simulink model "NonIsolatedDCDCTestHarnessPlant"  (R2026a)
settings: Solver=ode23t  StopTime=0.02  MaxStep=1e-5  AbsTol=1e-3
PreLoadFcn:
  | NonIsolatedDCDCDefaultInputParameters;
model workspace (MAT data in the model file):
  ConverterKey = "NonIsolatedDCDC"
undefined symbols (not defined in the file or in its folder): DiscIntNeverNeededParam, nonIsolatedDCDCController
libraries: nesl_utility x47, ee_lib x43, fl_lib x42
(part 1 of 5)
settings Model: Creator=vsolaise  LastModifiedBy=vsolaise
settings SimscapeCC: SimscapeNominalValues="[{\"value\":\"1\",\"unit\":\"A\"},{\"value\":\"1\",\"unit\":\"bar\"},{\"value\":\"1\",\"unit\":\"cm^2\"},{\"value\":\"1\",\"unit\":\"cm^3/s\"},{\"value\":\"1\",\"unit\":\"kJ/kg\"},{\"value\":\"1\",\"unit\":\"kW\"},{\"value\":\"1\",\"unit\":\"l\"},{\"value\":\"1\",\"unit\":\"N\"},{\"value\":\"1\",\"unit\":\"N*m\"},{\"value\":\"1\",\"unit\":\"V\"}]"  SimscapeLogDataHistory=5000.0

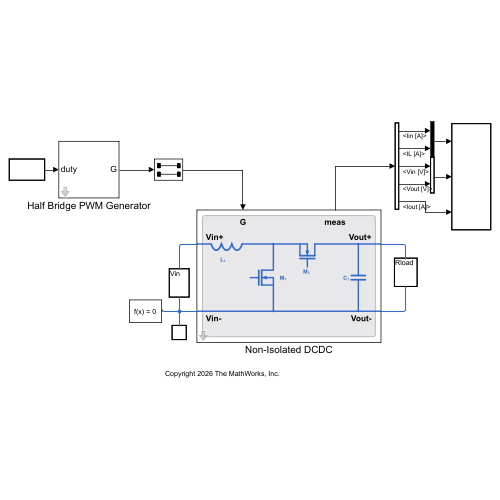
[thumbnail: Simulink's stored preview of the top-level diagram]
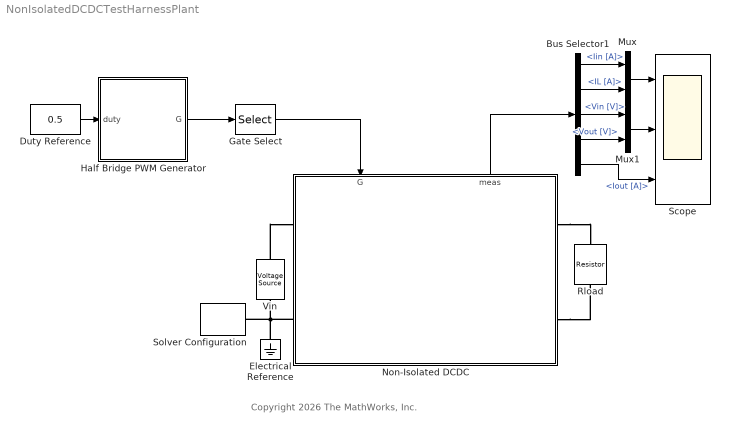
== system NonIsolatedDCDCTestHarnessPlant ==
  note: Copyright 2026 The MathWorks, Inc.
  Bus Selector1 : BusSelector  OutputSignals=Iin [A],IL [A],Vin [V],Vout [V],Iout [A]
  Duty Reference : Constant  Value=0.5
  Electrical Reference : fl_lib/Electrical/Electrical Elements/Electrical Reference
  Gate Select : Selector  InputPortWidth=2  IndexOptions=Index vector (dialog)  Indices=[1 2]  OutputSizes=1
  Half Bridge PWM Generator : Subsystem  mask(Half Bridge PWM Generator){solverMode=Variable-step (continuous), Ts=1e-8, Fsw=nonIsolatedDCDCController.Fsw.value, Tdead=nonIsolatedDCDCController.Tdead.value, gateVoltageOn=nonIsolatedDCDCController.gateVoltageOn.value, gateVoltageOff=nonIsolatedDCDCController.gateVoltageOff.value}
      mask prompts: solverMode "Solver mode"; Ts "Sample time (s)"; Fsw "Switching frequency (Hz)"; Tdead "Dead time (s)"; gateVoltageOn "Gate ON voltage (V)"; gateVoltageOff "Gate OFF voltage (V)"
      mask help:
      | This block generates half-bridge PWM gate signals with a dead time from a commanded duty cycle.
      |
      | For a variable-step solver, set Solver mode to Variable-step (continuous). For a fixed-step solver, set Solver mode to Fixed-step (discrete) and set Sample time to a positive value.
      mask init:
      | % Solver mode. Switch every sawtooth ramp in this block between its continuous
      | % and its discrete implementation, and show the sample time only when it is used.
      | pwmGeneratorBlock = gcb;
      | if strcmp(get_param(pwmGeneratorBlock, 'solverMode'), 'Fixed-step (discrete)')
      |     pwmGeneratorRampChoice = 'FixedStep';
      |     pwmGeneratorSampleTimeVisibility = 'on';
      | else
      |     pwmGeneratorRampChoice = 'VariableStep';
      |     pwmGeneratorSampleTimeVisibility = 'off';
      | end
      | 
      | % A block may hold more than one ramp, at any depth, so the ramps are found by the
      | % "Ramp Mode" suffix on their names rather than by one fixed path. The match filter
      | % keeps every variant choice in the search, which is also what silences the
      | % find_system default-variants warning.
      | pwmGeneratorRamps = find_system(pwmGeneratorBlock, ...
      |     'MatchFilter', @Simulink.match.allVariants, 'LookUnderMasks', 'all', ...
      |     'FollowLinks', 'on', 'Regexp', 'on', 'BlockType', 'SubSystem', ...
      |     'Name', 'Ramp Mode$');
      | for pwmGeneratorRampIndex = 1:numel(pwmGeneratorRamps)
      |     set_param(pwmGeneratorRamps{pwmGeneratorRampIndex}, ...
      |         'LabelModeActiveChoice', pwmGeneratorRampChoice);
      | end
      | 
      | % Only the discrete ramp declares a rate, so the sample time is hidden in the
      | % continuous mode. The guard keeps the code silent on a mask still being built.
      | pwmGeneratorMask = Simulink.Mask.get(pwmGeneratorBlock);
      | pwmGeneratorSampleTime = pwmGeneratorMask.getParameter('Ts');
      | if ~isempty(pwmGeneratorSampleTime)
      |     pwmGeneratorSampleTime.Visible = pwmGeneratorSampleTimeVisibility;
      | end
      mask Help: web('HalfBridgePWMGenerator.html')
      mask TypeOptions solverMode: Variable-step (continuous) | Fixed-step (discrete)
      mask Callback solverMode:
      | % Solver mode. Switch every sawtooth ramp in this block between its continuous
      | % and its discrete implementation, and show the sample time only when it is used.
      | pwmGeneratorBlock = gcb;
      | if strcmp(get_param(pwmGeneratorBlock, 'solverMode'), 'Fixed-step (discrete)')
      |     pwmGeneratorRampChoice = 'FixedStep';
      |     pwmGeneratorSampleTimeVisibility = 'on';
      | else
      |     pwmGeneratorRampChoice = 'VariableStep';
      |     pwmGeneratorSampleTimeVisibility = 'off';
      | end
      | 
      | % A block may hold more than one ramp, at any depth, so the ramps are found by the
      | % "Ramp Mode" suffix on their names rather than by one fixed path. The match filter
      | % keeps every variant choice in the search, which is also what silences the
      | % find_system default-variants warning.
      | pwmGeneratorRamps = find_system(pwmGeneratorBlock, ...
      |     'MatchFilter', @Simulink.match.allVariants, 'LookUnderMasks', 'all', ...
      |     'FollowLinks', 'on', 'Regexp', 'on', 'BlockType', 'SubSystem', ...
      |     'Name', 'Ramp Mode$');
      | for pwmGeneratorRampIndex = 1:numel(pwmGeneratorRamps)
      |     set_param(pwmGeneratorRamps{pwmGeneratorRampIndex}, ...
      |         'LabelModeActiveChoice', pwmGeneratorRampChoice);
      | end
      | 
      | % Only the discrete ramp declares a rate, so the sample time is hidden in the
      | % continuous mode. The guard keeps the code silent on a mask still being built.
      | pwmGeneratorMask = Simulink.Mask.get(pwmGeneratorBlock);
      | pwmGeneratorSampleTime = pwmGeneratorMask.getParameter('Ts');
      | if ~isempty(pwmGeneratorSampleTime)
      |     pwmGeneratorSampleTime.Visible = pwmGeneratorSampleTimeVisibility;
      | end
      mask DialogControl DescTextVar Prompt:
      | This block generates half-bridge PWM gate signals with a dead time from a commanded duty cycle.
      | 
      | For a variable-step solver, set Solver mode to Variable-step (continuous). For a fixed-step solver, set Solver mode to Fixed-step (discrete) and set Sample time to a positive value.
      mask DialogControl SolverPanel Prompt: Solver Settings
      mask DialogControl SwitchingPanel Prompt: Switching Parameters
      mask DialogControl GateDrivePanel Prompt: Gate Drive
  Mux : Mux  Inputs=2
  Mux1 : Mux  Inputs=2
  Non-Isolated DCDC : Subsystem  mask(Non-Isolated DC-DC Converter){modelOption=Synchronous Boost, ratedPower=1500, ratedPower_unit=W, Vin=200, Vin_unit=V, Vout=400, Vout_unit=V, Fsw=100000, Fsw_unit=Hz, L=4.356e-4, L_unit=H, RL=0.05, RL_unit=Ohm, C=1.8651e-4, C_unit=F, Rco=0.02, Rco_unit=Ohm, Vco=320, Vco_unit=V, switchDeviceOption=MOSFET (Ideal, Switching) with Thermal, RdsOn=0.02, RdsOn_unit=Ohm, GdsOff=1e-8, GdsOff_unit=1/Ohm, Vth=0.5, Vth_unit=V, VfBody=2.04, VfBody_unit=V, RdBody=0.004, RdBody_unit=Ohm, GdBody=1e-6, GdBody_unit=1/Ohm, diodeDeviceOption=Ideal Diode, Vf=0.5, Vf_unit=V, Rd=0.01, Rd_unit=Ohm, Gd=1e-8, Gd_unit=1/Ohm, simTemp=25, simTemp_unit=degC}
      mask prompts: modelOption "Topology"; ratedPower "Rated power"; Vin "Input voltage"; Vout "Output voltage"; Fsw "Switching frequency"; L "Inductance"; RL "Inductor resistance"; C "Output capacitance"; Rco "Capacitor ESR"; Vco "Initial output capacitor voltage"; switchDeviceOption "Main switch device"; RdsOn "On-state resistance"; GdsOff "Off-state conductance"; Vth "Threshold voltage"; VfBody "Body diode forward voltage"; RdBody "Body diode on resistance"; GdBody "Body diode off conductance"; diodeDeviceOption "Diode device"; Vf "Diode forward voltage"; Rd "Diode on resistance"; Gd "Diode off conductance"; simTemp "Simulation temperature"
      mask help: Buck, Boost, or Buck-Boost DC-DC converter with optional synchronous rectification
      mask init:
      | %% Unit conversion: convert displayed values to base SI units
      | convMap = containers.Map( ...
      |     {'W','kW','MW','V','kV','mV','F','mF','uF','nF','pF', ...
      |      'H','mH','uH','nH','Ohm','kOhm','mOhm','S','mS','1/Ohm', ...
      |      'Hz','kHz','MHz'}, ...
      |     {1, 1e3, 1e6, 1, 1e3, 1e-3, 1, 1e-3, 1e-6, 1e-9, 1e-12, ...
      |      1, 1e-3, 1e-6, 1e-9, 1, 1e3, 1e-3, 1, 1e-3, 1, ...
      |      1, 1e3, 1e6});
      | 
      | ratedPower_SI = ratedPower * convMap(ratedPower_unit);
      | Vin_SI = Vin * convMap(Vin_unit);
      | Vout_SI = Vout * convMap(Vout_unit);
      | Fsw_SI = Fsw * convMap(Fsw_unit);
      | L_SI = L * convMap(L_unit);
      | RL_SI = RL * convMap(RL_unit);
      | C_SI = C * convMap(C_unit);
      | Rco_SI = Rco * convMap(Rco_unit);
      | Vco_SI = Vco * convMap(Vco_unit);
      | RdsOn_SI = RdsOn * convMap(RdsOn_unit);
      | GdsOff_SI = GdsOff * convMap(GdsOff_unit);
      | Vth_SI = Vth * convMap(Vth_unit);
      | Vf_SI = Vf * convMap(Vf_unit);
      | Rd_SI = Rd * convMap(Rd_unit);
      | Gd_SI = Gd * convMap(Gd_unit);
      | VfBody_SI = VfBody * convMap(VfBody_unit);
      | RdBody_SI = RdBody * convMap(RdBody_unit);
      | GdBody_SI = GdBody * convMap(GdBody_unit);
      | 
      | %% Simulation temperature
      | % Temperature is an offset unit (K = degC + 273.15), so it cannot use convMap.
      | % simTemp_K is read by the thermal MOSFET junction target and Temperature Source,
      | % and by the tabulated diode device temperature.
      | if strcmp(simTemp_unit, 'degC')
      |     simTemp_K = simTemp + 273.15;
      | else
      |     simTemp_K = simTemp;
      | end
      | 
      | %% Apply variant selection
      | selectDCDCModelOption(gcb);
      settings: CopyFcn="set_param(gcbh,\"LinkStatus\",\"none\");"  PortSchema="{\"entries\":[{\"content\":{\"sides\":[{\"content\":{\"connectorIds\":[\"LConn1\",\"LConn2\"]},\"type\":\"ConnectorPlacement.EquallySpacedRectSide\",\"uuid\":\"902a8dfc-7104-4c05-856d-94df839e3447\"},{\"content\":{\"connectorIds\":[\"RConn1\",\"RConn2\"],\"side\":\"RIGHT\"},\"type\":\"ConnectorPlacement.EquallySpacedRectSide\",\"uuid\":\"60097652-723c-4c8b-adb2-e2e896cce9b8\"},{\"content\":{\"connectorIds\":[\"In1\",\"Out1\"],\"side\":\"TOP\"},\"type\":\"ConnectorPlacement.EquallySpacedRectSide\",\"uuid\":\"37713e19-e822-434b-b66d-56986e674464\"}]},\"type\":\"ConnectorPlacement.EquallySpacedConnector\",\"uuid\":\"e0b4e08f-2e15-4704-9b91-0fcfb097a2d4\"}],\"packageUris\":[\"http://schema.mathworks.com/mf0/Connector/R2020b\"],\"version\":\"1.0\"}"
      mask Help: web('NonIsolatedDCDC.html')
      mask TypeOptions modelOption: Buck | Synchronous Buck | Boost | Synchronous Boost | Buck-Boost | Synchronous Buck-Boost
      mask Callback modelOption: selectDCDCModelOption(gcb);
      mask TypeOptions ratedPower_unit: W | kW | MW
      mask TypeOptions Vin_unit: V | mV | kV
      mask TypeOptions Vout_unit: V | mV | kV
      mask TypeOptions Fsw_unit: Hz | kHz | MHz
      mask TypeOptions L_unit: H | mH | uH | nH
      mask TypeOptions RL_unit: Ohm | mOhm
      mask TypeOptions C_unit: F | mF | uF | nF | pF
      mask TypeOptions Rco_unit: Ohm | mOhm
      mask TypeOptions Vco_unit: V | kV | mV
      mask TypeOptions switchDeviceOption: Ideal Switch | MOSFET (Ideal, Switching) with Thermal
      mask Callback switchDeviceOption: selectDCDCMainSwitch(gcb);
      mask TypeOptions RdsOn_unit: Ohm | mOhm
      mask TypeOptions GdsOff_unit: 1/Ohm | S
      mask TypeOptions Vth_unit: V | mV
      mask TypeOptions VfBody_unit: V | mV
      mask TypeOptions RdBody_unit: Ohm | mOhm
      mask TypeOptions GdBody_unit: 1/Ohm | S
      mask TypeOptions diodeDeviceOption: Ideal Diode | Tabulated Diode
      mask Callback diodeDeviceOption: selectDCDCDiodeDevice(gcb);
      mask TypeOptions Vf_unit: V | mV
      mask TypeOptions Rd_unit: Ohm | mOhm
      mask TypeOptions Gd_unit: 1/Ohm | S
      mask TypeOptions simTemp_unit: degC | K
      mask DialogControl DC_DCConverterParameters Prompt: DC-DC Converter Parameters
      mask DialogControl SwitchDevice Prompt: Switch Device
      mask DialogControl openMOSFETMask Prompt: Open MOSFET block mask
      mask DialogControl openMOSFETMask Callback: openDCDCMOSFETMask(gcb);
      mask DialogControl DiodeDevice Prompt: Diode Device
      mask DialogControl openDiodeMask Prompt: Open Diode block mask
      mask DialogControl openDiodeMask Callback: openDCDCDiodeMask(gcb);
      mask DialogControl ExportPanel Prompt: Export to Unmasked Subsystem
      mask DialogControl ExportInfo Prompt: To customize the converter, export it as an unmasked subsystem with the active variant flattened - a standalone, fully-editable circuit plus a parameter file. Requires the "Variant Manager for Simulink" add-on.
      mask DialogControl exportToModel Prompt: Export
      mask DialogControl exportToModel Callback: exportConverterModelFromMask(gcb);
      mask Display:
      | topology = get_param(gcb, 'modelOption');
      | if strcmp(topology, 'Buck')
      |     image('BuckDiodeIcon.svg');
      | elseif strcmp(topology, 'Synchronous Buck')
      |     image('BuckSyncMOSIcon.svg');
      | elseif strcmp(topology, 'Boost')
      |     image('BoostDiodeIcon.svg');
      | elseif strcmp(topology, 'Synchronous Boost')
      |     image('BoostSyncMOSIcon.svg');
      | elseif strcmp(topology, 'Buck-Boost')
      |     image('BuckBoostDiodeIcon.svg');
      | else
      |     image('BuckBoostSyncMOSIcon.svg');
      | end
  Rload : fl_lib/Electrical/Electrical Elements/Resistor  R=106.667 Ohm  i_specify=off  i_priority=None  i=0 A  i_nominal_specify=off  i_nominal_value=1  i_nominal_unit=A  v_specify=off  v_priority=None  v=0 V  v_nominal_specify=off  v_nominal_value=1  v_nominal_unit=V
  Scope : Scope  NumInputPorts=3
      settings: ActiveDisplayString=3  Title=Output Current (A)  ActiveDisplayYMinimum=2.82510959569979  ActiveDisplayYMaximum=4.5280130894318766
  Solver Configuration : nesl_utility/Solver Configuration  PhysicalDomain=network_engine_domain  SubClassName=solver  LeftPortType=input  RightPortType=generic  Tones=[]  Harmonics=[]  SimulateNoise=off  Profile=off  UseLocalSampling=off  EnableSwitchedLinearOptims=on  FrequencyDomain=off  UseCCode=off  RelTol=0.001  AbsTol=0.001  MinStep=1e-09  ToWorkspace=off  RevertToSquareIcSolve=off  NumHomotopyIterations=100  PhasorMode=off  PhasorModeNumHarmonics=1  ConsistencySolver=NEWTON_XTOL_AFTER_FTOL  CanonicalOrdering=UNORDERED  OptimizeIntermediates=UNOPTIMIZED  IndexReductionMethod=DerivativeReplacement  DoDC=off  ResidualTolerance=1e-09  ConsistencyTolSource=GLOBAL  ConsistencyAbsTol=0.001  ConsistencyRelTol=0.001  ConsistencyTolFactor=0.001  UseLocalSolver=on  LocalSolverChoice=NE_BACKWARD_EULER_ADVANCER  ResolveIndetEquations=on  FunctionEvalNumThread=1  LocalSolverSampleTime=2e-7  DoFixedCost=on  MaxNonlinIter=3  MaxModeIter=2  ComputeImpulses=off  ImpulseIterations=2  LinearAlgebra=auto  LinearAlgebraNumThread=0  EquationFormulation=NE_TIME_EF  DelaysMemoryBudget=1024  AutomaticFiltering=on  FilteringTimeConstant=0.001  PartitionStorageMethod=AS_NEEDED  PartitionMemoryBudget=1024  PartitionMethod=ROBUST  MultibodyUseLocalSolver=off  MultibodyLocalSolverChoice=ODE1  MultibodyLocalSolverSampleTime=0.001
  Vin : ee_lib/Sources/Voltage Source  dc_voltage=200 V  ac_voltage=0 V  ac_shift=0 rad  ac_frequency=60 Hz  noise_mode=ee.enum.sources.noise.Disabled  PSD=0 V^2/Hz  sample_time=1e-3 s  repeatability=ee.enum.sources.repeatability.NotRepeatable  user_seed=0  auto_seed=4267928862  i_specify=off  i_priority=None  i=0 A  i_nominal_specify=off  i_nominal_value=1  i_nominal_unit=A  v_specify=off  v_priority=None  v=0 V  v_nominal_specify=off  v_nominal_value=1  v_nominal_unit=V
  wires:
  Non-Isolated DCDC/1(meas) -> Bus Selector1/1
  Bus Selector1/2 -> Mux/2  "<IL [A]>"
  Bus Selector1/1 -> Mux/1  "<Iin [A]>"
  Bus Selector1/3 -> Mux1/1  "<Vin [V]>"
  Bus Selector1/4 -> Mux1/2  "<Vout [V]>"
  Mux1/1 -> Scope/2
  Mux/1 -> Scope/1
  Bus Selector1/5 -> Scope/3  "<Iout [A]>"
  Duty Reference/1 -> Half Bridge PWM Generator/1(duty)
  Half Bridge PWM Generator/1(G) -> Gate Select/1
  Gate Select/1 -> Non-Isolated DCDC/1(G)
  connections:
  Vin/LConn1 -- Non-Isolated DCDC/LConn1
  Non-Isolated DCDC/RConn1 -- Rload/LConn1
  Non-Isolated DCDC/RConn2 -- Rload/RConn1
  Electrical Reference/LConn1 -- Solver Configuration/RConn1 -- Non-Isolated DCDC/LConn2 -- Vin/RConn1

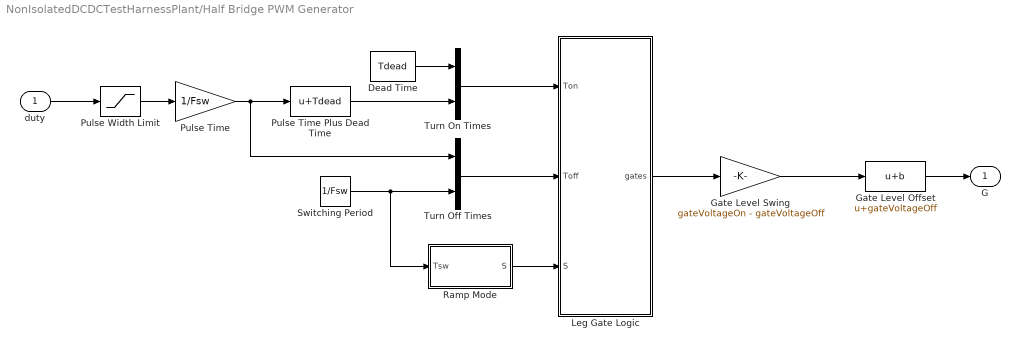
== system NonIsolatedDCDCTestHarnessPlant/Half Bridge PWM Generator ==
  duty : Inport
  Dead Time : Constant  Value=Tdead
  Gate Level Offset : Bias  Bias=gateVoltageOff
  Gate Level Swing : Gain  Gain=gateVoltageOn - gateVoltageOff
  Leg Gate Logic : Subsystem
  Pulse Time : Gain  Gain=1/Fsw
  Pulse Time Plus Dead Time : Bias  Bias=Tdead
  Pulse Width Limit : Saturate  UpperLimit=1 - Tdead*Fsw  LowerLimit=Tdead*Fsw
  Ramp Mode : Subsystem  Variant=on  VariantControlMode=label  LabelModeActiveChoice=VariableStep
  Switching Period : Constant  Value=1/Fsw
  Turn Off Times : Mux  Inputs=2
  Turn On Times : Mux  Inputs=2
  G : Outport
  wires:
  Gate Level Offset/1 -> G/1
  Leg Gate Logic/1(gates) -> Gate Level Swing/1
  Ramp Mode/1(S) -> Leg Gate Logic/3(S)
  Turn Off Times/1 -> Leg Gate Logic/2(Toff)
  Turn On Times/1 -> Leg Gate Logic/1(Ton)
  Gate Level Swing/1 -> Gate Level Offset/1
  Switching Period/1 -> Ramp Mode/1(Tsw), Turn Off Times/2
  Pulse Time Plus Dead Time/1 -> Turn On Times/2
  Dead Time/1 -> Turn On Times/1
  Pulse Time/1 -> Turn Off Times/1, Pulse Time Plus Dead Time/1
  Pulse Width Limit/1 -> Pulse Time/1
  duty/1 -> Pulse Width Limit/1

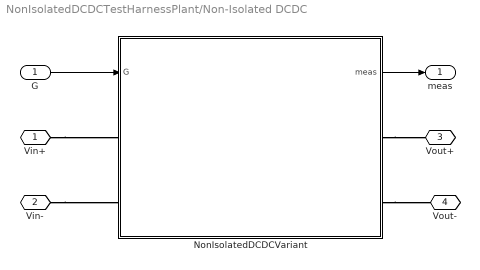
== system NonIsolatedDCDCTestHarnessPlant/Non-Isolated DCDC ==
  G : Inport
  NonIsolatedDCDCVariant : Subsystem  Variant=on  VariantControlMode=label  LabelModeActiveChoice=SynchronousBoost
  Vin+ : PMIOPort  Side=Left
  Vin- : PMIOPort  Port=2  Side=Left
  Vout+ : PMIOPort  Port=3  Side=Right
  Vout- : PMIOPort  Port=4  Side=Right
  meas : Outport
  wires:
  NonIsolatedDCDCVariant/1(meas) -> meas/1
  G/1 -> NonIsolatedDCDCVariant/1(G)
  connections:
  NonIsolatedDCDCVariant/RConn2 -- Vout-/RConn1
  NonIsolatedDCDCVariant/RConn1 -- Vout+/RConn1
  Vin-/RConn1 -- NonIsolatedDCDCVariant/LConn2
  Vin+/RConn1 -- NonIsolatedDCDCVariant/LConn1

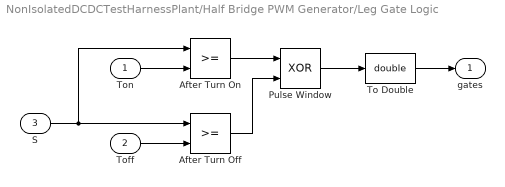
== system NonIsolatedDCDCTestHarnessPlant/Half Bridge PWM Generator/Leg Gate Logic ==
  Ton : Inport
  Toff : Inport  Port=2
  S : Inport  Port=3
  After Turn Off : RelationalOperator
  After Turn On : RelationalOperator
  Pulse Window : Logic  Operator=XOR
  To Double : DataTypeConversion  OutDataTypeStr=double
  gates : Outport
  wires:
  To Double/1 -> gates/1
  Pulse Window/1 -> To Double/1
  After Turn Off/1 -> Pulse Window/2
  After Turn On/1 -> Pulse Window/1
  S/1 -> After Turn On/1, After Turn Off/1
  Toff/1 -> After Turn Off/2
  Ton/1 -> After Turn On/2

== system NonIsolatedDCDCTestHarnessPlant/Half Bridge PWM Generator/Ramp Mode ==
  Tsw : Inport
  FixedStep : Subsystem  VariantControl=FixedStep
  VariableStep : Subsystem  VariantControl=VariableStep
  S : Outport

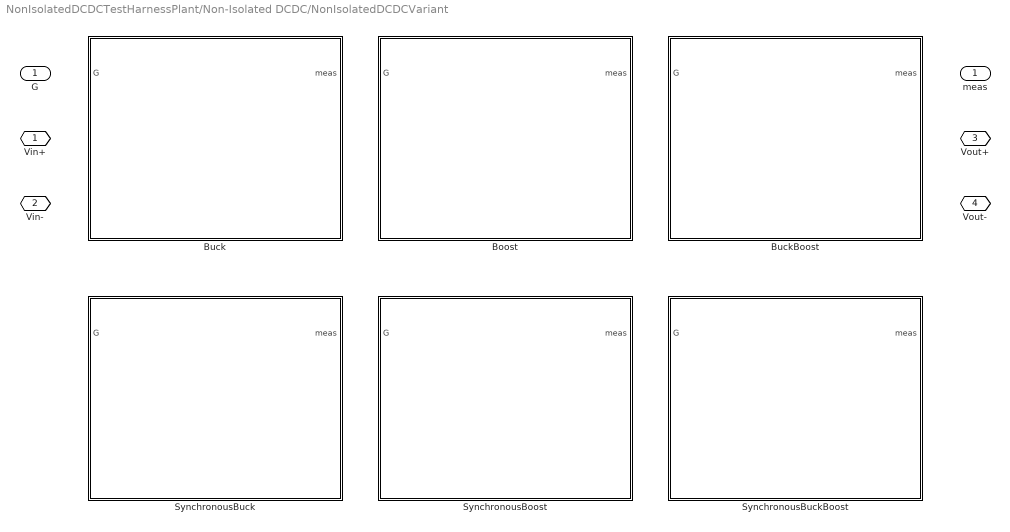
== system NonIsolatedDCDCTestHarnessPlant/Non-Isolated DCDC/NonIsolatedDCDCVariant ==
  G : Inport
  Boost : Subsystem  VariantControl=Boost
  Buck : Subsystem  VariantControl=Buck
  BuckBoost : Subsystem  VariantControl=BuckBoost
  SynchronousBoost : Subsystem  VariantControl=SynchronousBoost
  SynchronousBuck : Subsystem  VariantControl=SynchronousBuck
  SynchronousBuckBoost : Subsystem  VariantControl=SynchronousBuckBoost
  Vin+ : PMIOPort  Side=Left
  Vin- : PMIOPort  Port=2  Side=Left
  Vout+ : PMIOPort  Port=3  Side=Right
  Vout- : PMIOPort  Port=4  Side=Right
  meas : Outport

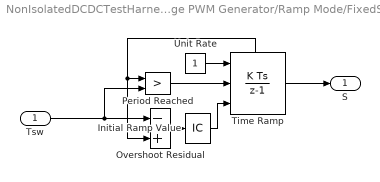
== system NonIsolatedDCDCTestHarnessPlant/Half Bridge PWM Generator/Ramp Mode/FixedStep ==
  Tsw : Inport
  Initial Ramp Value : InitialCondition  Value=0
  Overshoot Residual : Sum  Inputs=-+
  Period Reached : RelationalOperator  Operator=>  ZeroCross=off
  Time Ramp : DiscreteIntegrator  ExternalReset=rising  InitialConditionSource=external  SampleTime=Ts  ShowStatePort=on  ICPrevOutput=DiscIntNeverNeededParam  ICPrevScaledInput=DiscIntNeverNeededParam
  Unit Rate : Constant
  S : Outport
  wires:
  Initial Ramp Value/1 -> Time Ramp/3
  Overshoot Residual/1 -> Initial Ramp Value/1
  Time Ramp/State -> Overshoot Residual/2, Period Reached/1
  Tsw/1 -> Period Reached/2, Overshoot Residual/1
  Time Ramp/1 -> S/1
  Period Reached/1 -> Time Ramp/2
  Unit Rate/1 -> Time Ramp/1

== system NonIsolatedDCDCTestHarnessPlant/Half Bridge PWM Generator/Ramp Mode/VariableStep ==
  Tsw : Inport
  Initial Ramp Value : InitialCondition  Value=0
  Overshoot Residual : Sum  Inputs=-+
  Period Reached : RelationalOperator  Operator=>
  Time Ramp : Integrator  ExternalReset=rising  InitialConditionSource=external  ShowStatePort=on
  Unit Rate : Constant
  S : Outport
  wires:
  Initial Ramp Value/1 -> Time Ramp/3
  Overshoot Residual/1 -> Initial Ramp Value/1
  Time Ramp/State -> Overshoot Residual/2, Period Reached/1
  Tsw/1 -> Period Reached/2, Overshoot Residual/1
  Time Ramp/1 -> S/1
  Period Reached/1 -> Time Ramp/2
  Unit Rate/1 -> Time Ramp/1

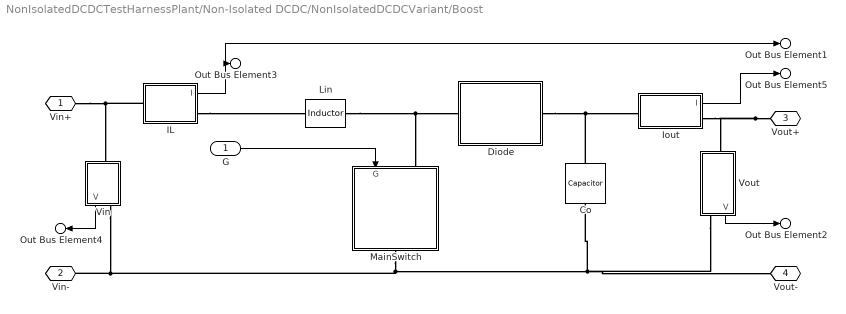
== system NonIsolatedDCDCTestHarnessPlant/Non-Isolated DCDC/NonIsolatedDCDCVariant/Boost ==
  G : Inport
  Co : ee_lib/Passive/Capacitor  cap_option=ee.enum.passive.capacitor.capOption.const  c=C_SI F  Cvec=[1e-05, 1e-06] F  Vvec=[0, 10] V  CV_table_symmetry=ee.enum.passive.capacitor.tableSymmetry.yes  f_vec=[1, 10] kHz  DFext_vec=[.8, 1.2]  enable_C_tol=ee.enum.toleranceApplication.none  averaging_period=0 s  C_tol=5  tol_distribution=ee.enum.toleranceDistribution.uniform  nSigma=4  r=Rco_SI Ohm  g=0 1/Ohm  enable_operating_limits=ee.enum.enable.no  operating_limit_action=ee.enum.passive.reportOpLim.warn  max_working_voltage_range=[-25, 25] V  power_rating=1 W  maxTemperature=85 degC  thermalEnable=false  thermalMass=1 J/K  i_specify=off  i_priority=None  i=0 A  i_nominal_specify=off  i_nominal_value=1  i_nominal_unit=A  v_specify=off  v_priority=None  v=0 V  v_nominal_specify=off  v_nominal_value=1  v_nominal_unit=V  vc_specify=on  vc_priority=High  vc=Vco_SI V  vc_nominal_specify=off  vc_nominal_value=1  vc_nominal_unit=V  T_specify=off  T_priority=None  T=298.15 K  T_nominal_specify=off  T_nominal_value=1  T_nominal_unit=K
  Diode : Subsystem  Variant=on  VariantControlMode=label  LabelModeActiveChoice=IdealDiode
  IL : Subsystem
      mask Display: disp('I')
  Iout : Subsystem
      mask Display: disp('I')
  Lin : ee_lib/Passive/Inductor  l=L_SI H  enable_L_tol=ee.enum.toleranceApplication.none  L_tol=20  tol_distribution=ee.enum.toleranceDistribution.uniform  nSigma=4  r=RL_SI Ohm  g=1e-9 1/Ohm  enable_operating_limits=ee.enum.enable.no  operating_limit_action=ee.enum.passive.reportOpLim.warn  max_working_current=1 A  power_rating=1 W  i_L_specify=off  i_L_priority=High  i_L=0 A  i_L_nominal_specify=off  i_L_nominal_value=1  i_L_nominal_unit=A
  MainSwitch : Subsystem  Variant=on  VariantControlMode=label  LabelModeActiveChoice=SwitchingMOSFETwithThermal
  Vin : Subsystem
      mask Display: disp('V')
  Vout : Subsystem
      settings: PortSchema="{\"entries\":[{\"content\":{\"sides\":[{\"content\":{\"connectorIds\":[\"LConn1\"]},\"type\":\"ConnectorPlacement.EquallySpacedRectSide\",\"uuid\":\"5f92137b-4b58-46b8-a68f-d3527484291c\"},{\"content\":{\"connectorIds\":[\"RConn1\",\"Out1\"],\"side\":\"RIGHT\"},\"type\":\"ConnectorPlacement.EquallySpacedRectSide\",\"uuid\":\"154b36f0-aa4a-4375-80c2-9c55af429c32\"},{\"content\":{\"side\":\"TOP\"},\"type\":\"ConnectorPlacement.EquallySpacedRectSide\",\"uuid\":\"6e01dd2b-817e-4c7e-a9bf-e017a248a3a8\"}]},\"type\":\"ConnectorPlacement.EquallySpacedConnector\",\"uuid\":\"a9d15cc4-68aa-466b-9599-7a273210f999\"}],\"packageUris\":[\"http://schema.mathworks.com/mf0/Connector/R2020b\"],\"version\":\"1.0\"}"
      mask Display: disp('V')
  Vin+ : PMIOPort  Side=Left
  Vin- : PMIOPort  Port=2  Side=Left
  Vout+ : PMIOPort  Port=3  Side=Right
  Vout- : PMIOPort  Port=4  Side=Right
  Out Bus Element1 : Outport  PortName=meas  Element=IL [A]
  Out Bus Element2 : Outport  PortName=meas  Element=Vout [V]
  Out Bus Element3 : Outport  PortName=meas  Element=Iin [A]
  Out Bus Element4 : Outport  PortName=meas  Element=Vin [V]
  Out Bus Element5 : Outport  PortName=meas  Element=Iout [A]
  wires:
  Vout/1(V) -> Out Bus Element2/1
  IL/1(I) -> Out Bus Element1/1, Out Bus Element3/1
  Vin/1(V) -> Out Bus Element4/1
  Iout/1(I) -> Out Bus Element5/1
  G/1 -> MainSwitch/1(G)
  connections:
  Vin+/RConn1 -- Vin/LConn1 -- IL/LConn1
  IL/RConn1 -- Lin/LConn1
  Vout+/RConn1 -- Iout/RConn1 -- Vout/LConn1
  MainSwitch/RConn1 -- Co/RConn1 -- Vout-/RConn1 -- Vout/RConn1 -- Vin-/RConn1 -- Vin/RConn1
  Lin/RConn1 -- MainSwitch/LConn1 -- Diode/LConn1
  Diode/RConn1 -- Co/LConn1 -- Iout/LConn1

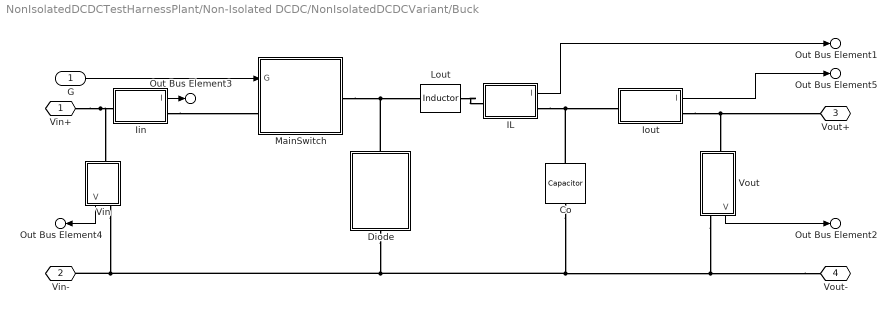
== system NonIsolatedDCDCTestHarnessPlant/Non-Isolated DCDC/NonIsolatedDCDCVariant/Buck ==
  G : Inport
  Co : ee_lib/Passive/Capacitor  cap_option=ee.enum.passive.capacitor.capOption.const  c=C_SI F  Cvec=[1e-05, 1e-06] F  Vvec=[0, 10] V  CV_table_symmetry=ee.enum.passive.capacitor.tableSymmetry.yes  f_vec=[1, 10] kHz  DFext_vec=[.8, 1.2]  enable_C_tol=ee.enum.toleranceApplication.none  averaging_period=0 s  C_tol=5  tol_distribution=ee.enum.toleranceDistribution.uniform  nSigma=4  r=Rco_SI Ohm  g=0 1/Ohm  enable_operating_limits=ee.enum.enable.no  operating_limit_action=ee.enum.passive.reportOpLim.warn  max_working_voltage_range=[-25, 25] V  power_rating=1 W  maxTemperature=85 degC  thermalEnable=false  thermalMass=1 J/K  i_specify=off  i_priority=None  i=0 A  i_nominal_specify=off  i_nominal_value=1  i_nominal_unit=A  v_specify=off  v_priority=None  v=0 V  v_nominal_specify=off  v_nominal_value=1  v_nominal_unit=V  vc_specify=on  vc_priority=High  vc=Vco_SI V  vc_nominal_specify=off  vc_nominal_value=1  vc_nominal_unit=V  T_specify=off  T_priority=None  T=298.15 K  T_nominal_specify=off  T_nominal_value=1  T_nominal_unit=K
  Diode : Subsystem  Variant=on  VariantControlMode=label  LabelModeActiveChoice=IdealDiode
  IL : Subsystem
      mask Display: disp('I')
  Iin : Subsystem
      mask Display: disp('I')
  Iout : Subsystem
      mask Display: disp('I')
  Lout : ee_lib/Passive/Inductor  l=L_SI H  enable_L_tol=ee.enum.toleranceApplication.none  L_tol=20  tol_distribution=ee.enum.toleranceDistribution.uniform  nSigma=4  r=RL_SI Ohm  g=1e-9 1/Ohm  enable_operating_limits=ee.enum.enable.no  operating_limit_action=ee.enum.passive.reportOpLim.warn  max_working_current=1 A  power_rating=1 W  i_L_specify=off  i_L_priority=High  i_L=0 A  i_L_nominal_specify=off  i_L_nominal_value=1  i_L_nominal_unit=A
  MainSwitch : Subsystem  Variant=on  VariantControlMode=label  LabelModeActiveChoice=SwitchingMOSFETwithThermal
  Vin : Subsystem
      mask Display: disp('V')
  Vout : Subsystem
      settings: PortSchema="{\"entries\":[{\"content\":{\"sides\":[{\"content\":{\"connectorIds\":[\"LConn1\"]},\"type\":\"ConnectorPlacement.EquallySpacedRectSide\",\"uuid\":\"5f92137b-4b58-46b8-a68f-d3527484291c\"},{\"content\":{\"connectorIds\":[\"RConn1\",\"Out1\"],\"side\":\"RIGHT\"},\"type\":\"ConnectorPlacement.EquallySpacedRectSide\",\"uuid\":\"154b36f0-aa4a-4375-80c2-9c55af429c32\"},{\"content\":{\"side\":\"TOP\"},\"type\":\"ConnectorPlacement.EquallySpacedRectSide\",\"uuid\":\"6e01dd2b-817e-4c7e-a9bf-e017a248a3a8\"}]},\"type\":\"ConnectorPlacement.EquallySpacedConnector\",\"uuid\":\"a9d15cc4-68aa-466b-9599-7a273210f999\"}],\"packageUris\":[\"http://schema.mathworks.com/mf0/Connector/R2020b\"],\"version\":\"1.0\"}"
      mask Display: disp('V')
  Vin+ : PMIOPort  Side=Left
  Vin- : PMIOPort  Port=2  Side=Left
  Vout+ : PMIOPort  Port=3  Side=Right
  Vout- : PMIOPort  Port=4  Side=Right
  Out Bus Element1 : Outport  PortName=meas  Element=IL [A]
  Out Bus Element2 : Outport  PortName=meas  Element=Vout [V]
  Out Bus Element3 : Outport  PortName=meas  Element=Iin [A]
  Out Bus Element4 : Outport  PortName=meas  Element=Vin [V]
  Out Bus Element5 : Outport  PortName=meas  Element=Iout [A]
  wires:
  IL/1(I) -> Out Bus Element1/1
  Vout/1(V) -> Out Bus Element2/1
  Iin/1(I) -> Out Bus Element3/1
  Vin/1(V) -> Out Bus Element4/1
  Iout/1(I) -> Out Bus Element5/1
  G/1 -> MainSwitch/1(G)
  connections:
  Iin/LConn1 -- Vin+/RConn1 -- Vin/LConn1
  Iin/RConn1 -- MainSwitch/LConn1
  Diode/RConn1 -- Lout/LConn1 -- MainSwitch/RConn1
  Lout/RConn1 -- IL/LConn1
  IL/RConn1 -- Iout/LConn1 -- Co/LConn1
  Iout/RConn1 -- Vout+/RConn1 -- Vout/LConn1
  Vout-/RConn1 -- Vout/RConn1 -- Vin-/RConn1 -- Vin/RConn1 -- Diode/LConn1 -- Co/RConn1

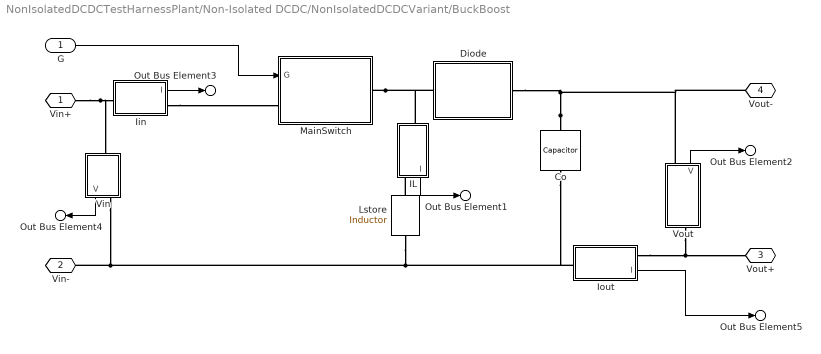
== system NonIsolatedDCDCTestHarnessPlant/Non-Isolated DCDC/NonIsolatedDCDCVariant/BuckBoost ==
  G : Inport
  Co : ee_lib/Passive/Capacitor  cap_option=ee.enum.passive.capacitor.capOption.const  c=C_SI F  Cvec=[1e-05, 1e-06] F  Vvec=[0, 10] V  CV_table_symmetry=ee.enum.passive.capacitor.tableSymmetry.yes  f_vec=[1, 10] kHz  DFext_vec=[.8, 1.2]  enable_C_tol=ee.enum.toleranceApplication.none  averaging_period=0 s  C_tol=5  tol_distribution=ee.enum.toleranceDistribution.uniform  nSigma=4  r=Rco_SI Ohm  g=0 1/Ohm  enable_operating_limits=ee.enum.enable.no  operating_limit_action=ee.enum.passive.reportOpLim.warn  max_working_voltage_range=[-25, 25] V  power_rating=1 W  maxTemperature=85 degC  thermalEnable=false  thermalMass=1 J/K  i_specify=off  i_priority=None  i=0 A  i_nominal_specify=off  i_nominal_value=1  i_nominal_unit=A  v_specify=off  v_priority=None  v=0 V  v_nominal_specify=off  v_nominal_value=1  v_nominal_unit=V  vc_specify=on  vc_priority=High  vc=Vco_SI V  vc_nominal_specify=off  vc_nominal_value=1  vc_nominal_unit=V  T_specify=off  T_priority=None  T=298.15 K  T_nominal_specify=off  T_nominal_value=1  T_nominal_unit=K
  Diode : Subsystem  Variant=on  VariantControlMode=label  LabelModeActiveChoice=IdealDiode
  IL : Subsystem
      settings: PortSchema="{\"entries\":[{\"content\":{\"sides\":[{\"content\":{\"connectorIds\":[\"LConn1\"]},\"type\":\"ConnectorPlacement.EquallySpacedRectSide\",\"uuid\":\"5f92137b-4b58-46b8-a68f-d3527484291c\"},{\"content\":{\"connectorIds\":[\"RConn1\",\"Out1\"],\"side\":\"RIGHT\"},\"type\":\"ConnectorPlacement.EquallySpacedRectSide\",\"uuid\":\"154b36f0-aa4a-4375-80c2-9c55af429c32\"},{\"content\":{\"side\":\"TOP\"},\"type\":\"ConnectorPlacement.EquallySpacedRectSide\",\"uuid\":\"6e01dd2b-817e-4c7e-a9bf-e017a248a3a8\"},{\"content\":{\"side\":\"BOTTOM\"},\"type\":\"ConnectorPlacement.EquallySpacedRectSide\",\"uuid\":\"8c02900b-7040-4e1d-af3e-df4ce1eee484\"}]},\"type\":\"ConnectorPlacement.EquallySpacedConnector\",\"uuid\":\"a9d15cc4-68aa-466b-9599-7a273210f999\"}],\"packageUris\":[\"http://schema.mathworks.com/mf0/Connector/R2020b\"],\"version\":\"1.0\"}"
      mask Display: disp('I')
  Iin : Subsystem
      mask Display: disp('I')
  Iout : Subsystem
      settings: PortSchema="{\"entries\":[{\"content\":{\"sides\":[{\"content\":{\"connectorIds\":[\"LConn1\"]},\"type\":\"ConnectorPlacement.EquallySpacedRectSide\",\"uuid\":\"7ec392cc-277f-44b1-b35e-7f2730db0397\"},{\"content\":{\"connectorIds\":[\"RConn1\",\"Out1\"],\"side\":\"RIGHT\"},\"type\":\"ConnectorPlacement.EquallySpacedRectSide\",\"uuid\":\"b0b5f2e0-1c59-4384-a465-885626d66149\"},{\"content\":{\"side\":\"TOP\"},\"type\":\"ConnectorPlacement.EquallySpacedRectSide\",\"uuid\":\"04ca4100-95ca-4157-98b9-4ff919847b2d\"}]},\"type\":\"ConnectorPlacement.EquallySpacedConnector\",\"uuid\":\"4f5cd1ed-b6ae-4123-b76e-0cf834717a23\"}],\"packageUris\":[\"http://schema.mathworks.com/mf0/Connector/R2020b\"],\"version\":\"1.0\"}"
      mask Display: disp('I')
  Lstore : ee_lib/Passive/Inductor  l=L_SI H  enable_L_tol=ee.enum.toleranceApplication.none  L_tol=20  tol_distribution=ee.enum.toleranceDistribution.uniform  nSigma=4  r=RL_SI Ohm  g=1e-9 1/Ohm  enable_operating_limits=ee.enum.enable.no  operating_limit_action=ee.enum.passive.reportOpLim.warn  max_working_current=1 A  power_rating=1 W  i_L_specify=off  i_L_priority=High  i_L=0 A  i_L_nominal_specify=off  i_L_nominal_value=1  i_L_nominal_unit=A
  MainSwitch : Subsystem  Variant=on  VariantControlMode=label  LabelModeActiveChoice=SwitchingMOSFETwithThermal
  Vin : Subsystem
      mask Display: disp('V')
  Vout : Subsystem
      settings: PortSchema="{\"entries\":[{\"content\":{\"sides\":[{\"content\":{\"connectorIds\":[\"LConn1\"]},\"type\":\"ConnectorPlacement.EquallySpacedRectSide\",\"uuid\":\"5f92137b-4b58-46b8-a68f-d3527484291c\"},{\"content\":{\"connectorIds\":[\"RConn1\",\"Out1\"],\"side\":\"RIGHT\"},\"type\":\"ConnectorPlacement.EquallySpacedRectSide\",\"uuid\":\"154b36f0-aa4a-4375-80c2-9c55af429c32\"},{\"content\":{\"side\":\"TOP\"},\"type\":\"ConnectorPlacement.EquallySpacedRectSide\",\"uuid\":\"6e01dd2b-817e-4c7e-a9bf-e017a248a3a8\"}]},\"type\":\"ConnectorPlacement.EquallySpacedConnector\",\"uuid\":\"a9d15cc4-68aa-466b-9599-7a273210f999\"}],\"packageUris\":[\"http://schema.mathworks.com/mf0/Connector/R2020b\"],\"version\":\"1.0\"}"
      mask Display: disp('V')
  Vin+ : PMIOPort  Side=Left
  Vin- : PMIOPort  Port=2  Side=Left
  Vout+ : PMIOPort  Port=3  Side=Right
  Vout- : PMIOPort  Port=4  Side=Right
  Out Bus Element1 : Outport  PortName=meas  Element=IL [A]
  Out Bus Element2 : Outport  PortName=meas  Element=Vout [V]
  Out Bus Element3 : Outport  PortName=meas  Element=Iin [A]
  Out Bus Element4 : Outport  PortName=meas  Element=Vin [V]
  Out Bus Element5 : Outport  PortName=meas  Element=Iout [A]
  wires:
  IL/1(I) -> Out Bus Element1/1
  Iin/1(I) -> Out Bus Element3/1
  Iout/1(I) -> Out Bus Element5/1
  Vin/1(V) -> Out Bus Element4/1
  Vout/1(V) -> Out Bus Element2/1
  G/1 -> MainSwitch/1(G)
  connections:
  Iout/RConn1 -- Vout/LConn1 -- Vout+/RConn1
  Iin/LConn1 -- Vin+/RConn1 -- Vin/LConn1
  Iin/RConn1 -- MainSwitch/LConn1
  Vin/RConn1 -- Vin-/RConn1 -- Iout/LConn1 -- Co/RConn1 -- Lstore/RConn1
  MainSwitch/RConn1 -- Diode/RConn1 -- IL/LConn1
  Lstore/LConn1 -- IL/RConn1
  Co/LConn1 -- Vout/RConn1 -- Vout-/RConn1 -- Diode/LConn1

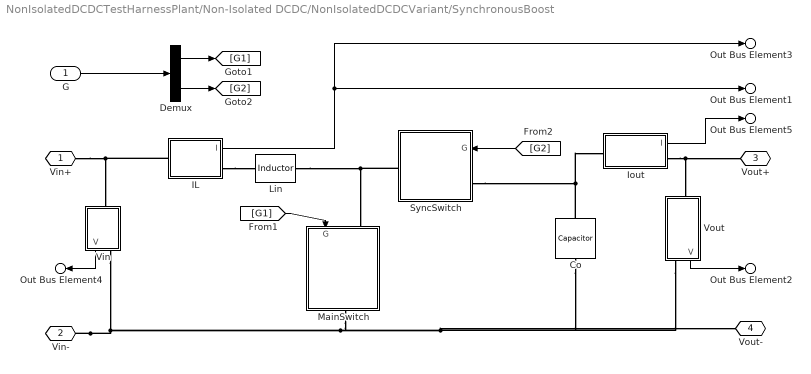
== system NonIsolatedDCDCTestHarnessPlant/Non-Isolated DCDC/NonIsolatedDCDCVariant/SynchronousBoost ==
  G : Inport
  Co : ee_lib/Passive/Capacitor  cap_option=ee.enum.passive.capacitor.capOption.const  c=C_SI F  Cvec=[1e-05, 1e-06] F  Vvec=[0, 10] V  CV_table_symmetry=ee.enum.passive.capacitor.tableSymmetry.yes  f_vec=[1, 10] kHz  DFext_vec=[.8, 1.2]  enable_C_tol=ee.enum.toleranceApplication.none  averaging_period=0 s  C_tol=5  tol_distribution=ee.enum.toleranceDistribution.uniform  nSigma=4  r=Rco_SI Ohm  g=0 1/Ohm  enable_operating_limits=ee.enum.enable.no  operating_limit_action=ee.enum.passive.reportOpLim.warn  max_working_voltage_range=[-25, 25] V  power_rating=1 W  maxTemperature=85 degC  thermalEnable=false  thermalMass=1 J/K  i_specify=off  i_priority=None  i=0 A  i_nominal_specify=off  i_nominal_value=1  i_nominal_unit=A  v_specify=off  v_priority=None  v=0 V  v_nominal_specify=off  v_nominal_value=1  v_nominal_unit=V  vc_specify=on  vc_priority=High  vc=Vco_SI V  vc_nominal_specify=off  vc_nominal_value=1  vc_nominal_unit=V  T_specify=off  T_priority=None  T=298.15 K  T_nominal_specify=off  T_nominal_value=1  T_nominal_unit=K
  Demux : Demux  Outputs=2
  IL : Subsystem
      mask Display: disp('I')
  Iout : Subsystem
      mask Display: disp('I')
  Lin : ee_lib/Passive/Inductor  l=L_SI H  enable_L_tol=ee.enum.toleranceApplication.none  L_tol=20  tol_distribution=ee.enum.toleranceDistribution.uniform  nSigma=4  r=RL_SI Ohm  g=1e-9 1/Ohm  enable_operating_limits=ee.enum.enable.no  operating_limit_action=ee.enum.passive.reportOpLim.warn  max_working_current=1 A  power_rating=1 W  i_L_specify=off  i_L_priority=High  i_L=0 A  i_L_nominal_specify=off  i_L_nominal_value=1  i_L_nominal_unit=A
  MainSwitch : Subsystem  Variant=on  VariantControlMode=label  LabelModeActiveChoice=SwitchingMOSFETwithThermal
  SyncSwitch : Subsystem  Variant=on  VariantControlMode=label  LabelModeActiveChoice=SwitchingMOSFETwithThermal
  Vin : Subsystem
      mask Display: disp('V')
  Vout : Subsystem
      settings: PortSchema="{\"entries\":[{\"content\":{\"sides\":[{\"content\":{\"connectorIds\":[\"LConn1\"]},\"type\":\"ConnectorPlacement.EquallySpacedRectSide\",\"uuid\":\"5f92137b-4b58-46b8-a68f-d3527484291c\"},{\"content\":{\"connectorIds\":[\"RConn1\",\"Out1\"],\"side\":\"RIGHT\"},\"type\":\"ConnectorPlacement.EquallySpacedRectSide\",\"uuid\":\"154b36f0-aa4a-4375-80c2-9c55af429c32\"},{\"content\":{\"side\":\"TOP\"},\"type\":\"ConnectorPlacement.EquallySpacedRectSide\",\"uuid\":\"6e01dd2b-817e-4c7e-a9bf-e017a248a3a8\"}]},\"type\":\"ConnectorPlacement.EquallySpacedConnector\",\"uuid\":\"a9d15cc4-68aa-466b-9599-7a273210f999\"}],\"packageUris\":[\"http://schema.mathworks.com/mf0/Connector/R2020b\"],\"version\":\"1.0\"}"
      mask Display: disp('V')
  Vin+ : PMIOPort  Side=Left
  Vin- : PMIOPort  Port=2  Side=Left
  Vout+ : PMIOPort  Port=3  Side=Right
  Vout- : PMIOPort  Port=4  Side=Right
  Out Bus Element1 : Outport  PortName=meas  Element=IL [A]
  Out Bus Element2 : Outport  PortName=meas  Element=Vout [V]
  Out Bus Element3 : Outport  PortName=meas  Element=Iin [A]
  Out Bus Element4 : Outport  PortName=meas  Element=Vin [V]
  Out Bus Element5 : Outport  PortName=meas  Element=Iout [A]
  wires:
  [G2] -> SyncSwitch/1(G)
  Demux/2 -> [G2]
  Demux/1 -> [G1]
  Iout/1(I) -> Out Bus Element5/1
  Vin/1(V) -> Out Bus Element4/1
  IL/1(I) -> Out Bus Element3/1, Out Bus Element1/1
  Vout/1(V) -> Out Bus Element2/1
  G/1 -> Demux/1
  [G1] -> MainSwitch/1(G)
  connections:
  Vin-/RConn1 -- Co/RConn1 -- Vout-/RConn1 -- Vout/RConn1 -- MainSwitch/RConn1 -- Vin/RConn1
  Iout/RConn1 -- Vout/LConn1 -- Vout+/RConn1
  IL/RConn1 -- Lin/LConn1
  Vin+/RConn1 -- IL/LConn1 -- Vin/LConn1
  SyncSwitch/RConn1 -- MainSwitch/LConn1 -- Lin/RConn1
  SyncSwitch/LConn1 -- Iout/LConn1 -- Co/LConn1

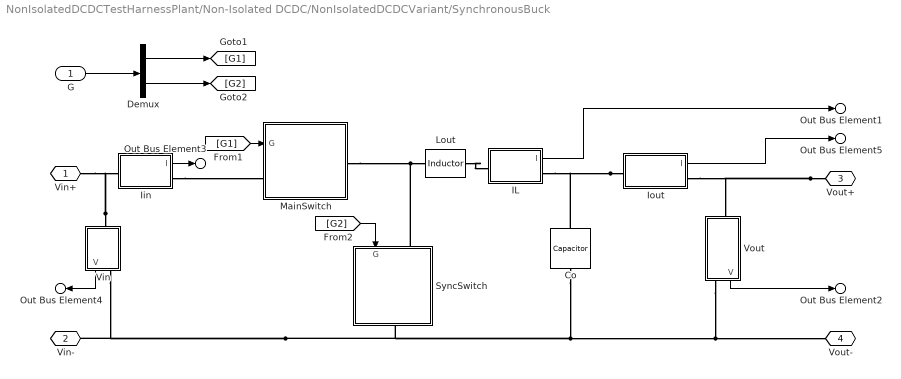
== system NonIsolatedDCDCTestHarnessPlant/Non-Isolated DCDC/NonIsolatedDCDCVariant/SynchronousBuck ==
  G : Inport
  Co : ee_lib/Passive/Capacitor  cap_option=ee.enum.passive.capacitor.capOption.const  c=C_SI F  Cvec=[1e-05, 1e-06] F  Vvec=[0, 10] V  CV_table_symmetry=ee.enum.passive.capacitor.tableSymmetry.yes  f_vec=[1, 10] kHz  DFext_vec=[.8, 1.2]  enable_C_tol=ee.enum.toleranceApplication.none  averaging_period=0 s  C_tol=5  tol_distribution=ee.enum.toleranceDistribution.uniform  nSigma=4  r=Rco_SI Ohm  g=0 1/Ohm  enable_operating_limits=ee.enum.enable.no  operating_limit_action=ee.enum.passive.reportOpLim.warn  max_working_voltage_range=[-25, 25] V  power_rating=1 W  maxTemperature=85 degC  thermalEnable=false  thermalMass=1 J/K  i_specify=off  i_priority=None  i=0 A  i_nominal_specify=off  i_nominal_value=1  i_nominal_unit=A  v_specify=off  v_priority=None  v=0 V  v_nominal_specify=off  v_nominal_value=1  v_nominal_unit=V  vc_specify=on  vc_priority=High  vc=Vco_SI V  vc_nominal_specify=off  vc_nominal_value=1  vc_nominal_unit=V  T_specify=off  T_priority=None  T=298.15 K  T_nominal_specify=off  T_nominal_value=1  T_nominal_unit=K
  Demux : Demux  Outputs=2
  IL : Subsystem
      mask Display: disp('I')
  Iin : Subsystem
      mask Display: disp('I')
  Iout : Subsystem
      mask Display: disp('I')
  Lout : ee_lib/Passive/Inductor  l=L_SI H  enable_L_tol=ee.enum.toleranceApplication.none  L_tol=20  tol_distribution=ee.enum.toleranceDistribution.uniform  nSigma=4  r=RL_SI Ohm  g=1e-9 1/Ohm  enable_operating_limits=ee.enum.enable.no  operating_limit_action=ee.enum.passive.reportOpLim.warn  max_working_current=1 A  power_rating=1 W  i_L_specify=off  i_L_priority=High  i_L=0 A  i_L_nominal_specify=off  i_L_nominal_value=1  i_L_nominal_unit=A
  MainSwitch : Subsystem  Variant=on  VariantControlMode=label  LabelModeActiveChoice=SwitchingMOSFETwithThermal
  SyncSwitch : Subsystem  Variant=on  VariantControlMode=label  LabelModeActiveChoice=SwitchingMOSFETwithThermal
  Vin : Subsystem
      mask Display: disp('V')
  Vout : Subsystem
      settings: PortSchema="{\"entries\":[{\"content\":{\"sides\":[{\"content\":{\"connectorIds\":[\"LConn1\"]},\"type\":\"ConnectorPlacement.EquallySpacedRectSide\",\"uuid\":\"5f92137b-4b58-46b8-a68f-d3527484291c\"},{\"content\":{\"connectorIds\":[\"RConn1\",\"Out1\"],\"side\":\"RIGHT\"},\"type\":\"ConnectorPlacement.EquallySpacedRectSide\",\"uuid\":\"154b36f0-aa4a-4375-80c2-9c55af429c32\"},{\"content\":{\"side\":\"TOP\"},\"type\":\"ConnectorPlacement.EquallySpacedRectSide\",\"uuid\":\"6e01dd2b-817e-4c7e-a9bf-e017a248a3a8\"}]},\"type\":\"ConnectorPlacement.EquallySpacedConnector\",\"uuid\":\"a9d15cc4-68aa-466b-9599-7a273210f999\"}],\"packageUris\":[\"http://schema.mathworks.com/mf0/Connector/R2020b\"],\"version\":\"1.0\"}"
      mask Display: disp('V')
  Vin+ : PMIOPort  Side=Left
  Vin- : PMIOPort  Port=2  Side=Left
  Vout+ : PMIOPort  Port=3  Side=Right
  Vout- : PMIOPort  Port=4  Side=Right
  Out Bus Element1 : Outport  PortName=meas  Element=IL [A]
  Out Bus Element2 : Outport  PortName=meas  Element=Vout [V]
  Out Bus Element3 : Outport  PortName=meas  Element=Iin [A]
  Out Bus Element4 : Outport  PortName=meas  Element=Vin [V]
  Out Bus Element5 : Outport  PortName=meas  Element=Iout [A]
  wires:
  Demux/2 -> [G2]
  Demux/1 -> [G1]
  Iout/1(I) -> Out Bus Element5/1
  Vin/1(V) -> Out Bus Element4/1
  Iin/1(I) -> Out Bus Element3/1
  Vout/1(V) -> Out Bus Element2/1
  IL/1(I) -> Out Bus Element1/1
  G/1 -> Demux/1
  [G1] -> MainSwitch/1(G)
  [G2] -> SyncSwitch/1(G)
  connections:
  Co/RConn1 -- Vout/RConn1 -- Vout-/RConn1 -- SyncSwitch/RConn1 -- Vin/RConn1 -- Vin-/RConn1
  Vout+/RConn1 -- Vout/LConn1 -- Iout/RConn1
  Iout/LConn1 -- IL/RConn1 -- Co/LConn1
  Lout/RConn1 -- IL/LConn1
  Lout/LConn1 -- SyncSwitch/LConn1 -- MainSwitch/RConn1
  Iin/RConn1 -- MainSwitch/LConn1
  Vin/LConn1 -- Vin+/RConn1 -- Iin/LConn1

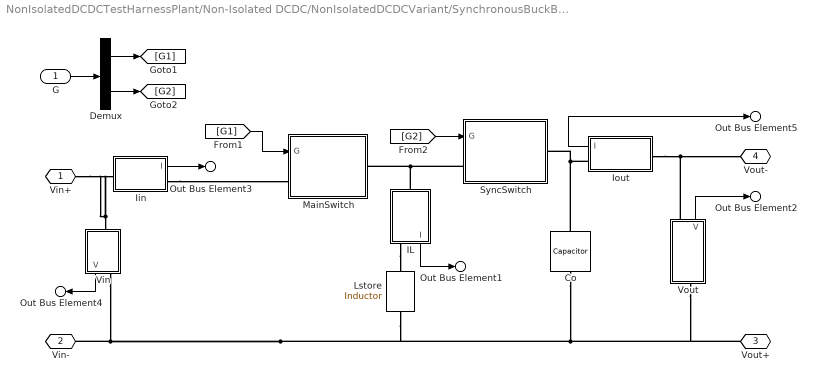
== system NonIsolatedDCDCTestHarnessPlant/Non-Isolated DCDC/NonIsolatedDCDCVariant/SynchronousBuckBoost ==
  G : Inport
  Co : ee_lib/Passive/Capacitor  cap_option=ee.enum.passive.capacitor.capOption.const  c=C_SI F  Cvec=[1e-05, 1e-06] F  Vvec=[0, 10] V  CV_table_symmetry=ee.enum.passive.capacitor.tableSymmetry.yes  f_vec=[1, 10] kHz  DFext_vec=[.8, 1.2]  enable_C_tol=ee.enum.toleranceApplication.none  averaging_period=0 s  C_tol=5  tol_distribution=ee.enum.toleranceDistribution.uniform  nSigma=4  r=Rco_SI Ohm  g=0 1/Ohm  enable_operating_limits=ee.enum.enable.no  operating_limit_action=ee.enum.passive.reportOpLim.warn  max_working_voltage_range=[-25, 25] V  power_rating=1 W  maxTemperature=85 degC  thermalEnable=false  thermalMass=1 J/K  i_specify=off  i_priority=None  i=0 A  i_nominal_specify=off  i_nominal_value=1  i_nominal_unit=A  v_specify=off  v_priority=None  v=0 V  v_nominal_specify=off  v_nominal_value=1  v_nominal_unit=V  vc_specify=on  vc_priority=High  vc=Vco_SI V  vc_nominal_specify=off  vc_nominal_value=1  vc_nominal_unit=V  T_specify=off  T_priority=None  T=298.15 K  T_nominal_specify=off  T_nominal_value=1  T_nominal_unit=K
  Demux : Demux  Outputs=2
  IL : Subsystem
      settings: PortSchema="{\"entries\":[{\"content\":{\"sides\":[{\"content\":{\"connectorIds\":[\"LConn1\"]},\"type\":\"ConnectorPlacement.EquallySpacedRectSide\",\"uuid\":\"5f92137b-4b58-46b8-a68f-d3527484291c\"},{\"content\":{\"connectorIds\":[\"RConn1\",\"Out1\"],\"side\":\"RIGHT\"},\"type\":\"ConnectorPlacement.EquallySpacedRectSide\",\"uuid\":\"154b36f0-aa4a-4375-80c2-9c55af429c32\"},{\"content\":{\"side\":\"TOP\"},\"type\":\"ConnectorPlacement.EquallySpacedRectSide\",\"uuid\":\"6e01dd2b-817e-4c7e-a9bf-e017a248a3a8\"}]},\"type\":\"ConnectorPlacement.EquallySpacedConnector\",\"uuid\":\"a9d15cc4-68aa-466b-9599-7a273210f999\"}],\"packageUris\":[\"http://schema.mathworks.com/mf0/Connector/R2020b\"],\"version\":\"1.0\"}"
      mask Display: disp('I')
  Iin : Subsystem
      mask Display: disp('I')
  Iout : Subsystem
      mask Display: disp('I')
  Lstore : ee_lib/Passive/Inductor  l=L_SI H  enable_L_tol=ee.enum.toleranceApplication.none  L_tol=20  tol_distribution=ee.enum.toleranceDistribution.uniform  nSigma=4  r=RL_SI Ohm  g=1e-9 1/Ohm  enable_operating_limits=ee.enum.enable.no  operating_limit_action=ee.enum.passive.reportOpLim.warn  max_working_current=1 A  power_rating=1 W  i_L_specify=off  i_L_priority=High  i_L=0 A  i_L_nominal_specify=off  i_L_nominal_value=1  i_L_nominal_unit=A
  MainSwitch : Subsystem  Variant=on  VariantControlMode=label  LabelModeActiveChoice=SwitchingMOSFETwithThermal
  SyncSwitch : Subsystem  Variant=on  VariantControlMode=label  LabelModeActiveChoice=SwitchingMOSFETwithThermal
  Vin : Subsystem
      mask Display: disp('V')
  Vout : Subsystem
      settings: PortSchema="{\"entries\":[{\"content\":{\"sides\":[{\"content\":{\"connectorIds\":[\"LConn1\"]},\"type\":\"ConnectorPlacement.EquallySpacedRectSide\",\"uuid\":\"5f92137b-4b58-46b8-a68f-d3527484291c\"},{\"content\":{\"connectorIds\":[\"RConn1\",\"Out1\"],\"side\":\"RIGHT\"},\"type\":\"ConnectorPlacement.EquallySpacedRectSide\",\"uuid\":\"154b36f0-aa4a-4375-80c2-9c55af429c32\"},{\"content\":{\"side\":\"TOP\"},\"type\":\"ConnectorPlacement.EquallySpacedRectSide\",\"uuid\":\"6e01dd2b-817e-4c7e-a9bf-e017a248a3a8\"}]},\"type\":\"ConnectorPlacement.EquallySpacedConnector\",\"uuid\":\"a9d15cc4-68aa-466b-9599-7a273210f999\"}],\"packageUris\":[\"http://schema.mathworks.com/mf0/Connector/R2020b\"],\"version\":\"1.0\"}"
      mask Display: disp('V')
  Vin+ : PMIOPort  Side=Left
  Vin- : PMIOPort  Port=2  Side=Left
  Vout+ : PMIOPort  Port=3  Side=Right
  Vout- : PMIOPort  Port=4  Side=Right
  Out Bus Element1 : Outport  PortName=meas  Element=IL [A]
  Out Bus Element2 : Outport  PortName=meas  Element=Vout [V]
  Out Bus Element3 : Outport  PortName=meas  Element=Iin [A]
  Out Bus Element4 : Outport  PortName=meas  Element=Vin [V]
  Out Bus Element5 : Outport  PortName=meas  Element=Iout [A]
  wires:
  Vout/1(V) -> Out Bus Element2/1
  Vin/1(V) -> Out Bus Element4/1
  Iout/1(I) -> Out Bus Element5/1
  Iin/1(I) -> Out Bus Element3/1
  Demux/2 -> [G2]
  Demux/1 -> [G1]
  G/1 -> Demux/1
  [G1] -> MainSwitch/1(G)
  [G2] -> SyncSwitch/1(G)
  IL/1(I) -> Out Bus Element1/1
  connections:
  Vin/RConn1 -- Co/RConn1 -- Vout+/RConn1 -- Vout/LConn1 -- Lstore/RConn1 -- Vin-/RConn1
  Vout/RConn1 -- Iout/LConn1 -- Vout-/RConn1
  Iin/RConn1 -- MainSwitch/LConn1
  Vin/LConn1 -- Vin+/RConn1 -- Iin/LConn1
  IL/LConn1 -- MainSwitch/RConn1 -- SyncSwitch/LConn1
  IL/RConn1 -- Lstore/LConn1
  Co/LConn1 -- SyncSwitch/RConn1 -- Iout/RConn1

== system NonIsolatedDCDCTestHarnessPlant/Non-Isolated DCDC/NonIsolatedDCDCVariant/Boost/Diode ==
  IdealDiode : Subsystem  VariantControl=IdealDiode
  TabulatedDiode : Subsystem  VariantControl=TabulatedDiode
  D : PMIOPort  Side=Left
  S : PMIOPort  Port=2  Side=Right

== system NonIsolatedDCDCTestHarnessPlant/Non-Isolated DCDC/NonIsolatedDCDCVariant/Boost/IL ==
  Current Sensor : fl_lib/Electrical/Electrical Sensors/Current Sensor
  PS-Simulink Converter : nesl_utility/PS-Simulink Converter  PhysicalDomain=network_engine_domain  SubClassName=ps_output  LeftPortType=input  RightPortType=output  PseudoPeriodic=off  Frequencies=[]  VectorFormat=inherit  Unit=inherit  AffineConversion=off
  + : PMIOPort  Side=Left
  - : PMIOPort  Port=2  Side=Right
  I : Outport
  wires:
  PS-Simulink Converter/1 -> I/1
  connections:
  Current Sensor/RConn1 -- PS-Simulink Converter/LConn1
  Current Sensor/RConn2 -- -/RConn1
  +/RConn1 -- Current Sensor/LConn1

== system NonIsolatedDCDCTestHarnessPlant/Non-Isolated DCDC/NonIsolatedDCDCVariant/Boost/Iout ==
  Current Sensor : fl_lib/Electrical/Electrical Sensors/Current Sensor
  PS-Simulink Converter : nesl_utility/PS-Simulink Converter  PhysicalDomain=network_engine_domain  SubClassName=ps_output  LeftPortType=input  RightPortType=output  PseudoPeriodic=off  Frequencies=[]  VectorFormat=inherit  Unit=inherit  AffineConversion=off
  + : PMIOPort  Side=Left
  - : PMIOPort  Port=2  Side=Right
  I : Outport
  wires:
  PS-Simulink Converter/1 -> I/1
  connections:
  Current Sensor/RConn1 -- PS-Simulink Converter/LConn1
  Current Sensor/RConn2 -- -/RConn1
  +/RConn1 -- Current Sensor/LConn1

== system NonIsolatedDCDCTestHarnessPlant/Non-Isolated DCDC/NonIsolatedDCDCVariant/Boost/MainSwitch ==
  G : Inport
  IdealSwitch : Subsystem  VariantControl=IdealSwitch
  SwitchingMOSFETwithThermal : Subsystem  VariantControl=SwitchingMOSFETwithThermal
  D : PMIOPort  Side=Left
  S : PMIOPort  Port=2  Side=Right

== system NonIsolatedDCDCTestHarnessPlant/Non-Isolated DCDC/NonIsolatedDCDCVariant/Boost/Vin ==
  PS-Simulink Converter : nesl_utility/PS-Simulink Converter  PhysicalDomain=network_engine_domain  SubClassName=ps_output  LeftPortType=input  RightPortType=output  PseudoPeriodic=off  Frequencies=[]  VectorFormat=inherit  Unit=inherit  AffineConversion=off
  Voltage Sensor : fl_lib/Electrical/Electrical Sensors/Voltage Sensor
  + : PMIOPort  Side=Left
  - : PMIOPort  Port=2  Side=Right
  V : Outport
  wires:
  PS-Simulink Converter/1 -> V/1
  connections:
  Voltage Sensor/RConn1 -- PS-Simulink Converter/LConn1
  Voltage Sensor/RConn2 -- -/RConn1
  +/RConn1 -- Voltage Sensor/LConn1

== system NonIsolatedDCDCTestHarnessPlant/Non-Isolated DCDC/NonIsolatedDCDCVariant/Boost/Vout ==
  PS-Simulink Converter : nesl_utility/PS-Simulink Converter  PhysicalDomain=network_engine_domain  SubClassName=ps_output  LeftPortType=input  RightPortType=output  PseudoPeriodic=off  Frequencies=[]  VectorFormat=inherit  Unit=inherit  AffineConversion=off
  Voltage Sensor : fl_lib/Electrical/Electrical Sensors/Voltage Sensor
  + : PMIOPort  Side=Left
  - : PMIOPort  Port=2  Side=Right
  V : Outport
  wires:
  PS-Simulink Converter/1 -> V/1
  connections:
  Voltage Sensor/RConn1 -- PS-Simulink Converter/LConn1
  Voltage Sensor/RConn2 -- -/RConn1
  +/RConn1 -- Voltage Sensor/LConn1

== system NonIsolatedDCDCTestHarnessPlant/Non-Isolated DCDC/NonIsolatedDCDCVariant/Buck/Diode ==
  IdealDiode : Subsystem  VariantControl=IdealDiode
  TabulatedDiode : Subsystem  VariantControl=TabulatedDiode
  D : PMIOPort  Side=Left
  S : PMIOPort  Port=2  Side=Right
